simulink model "nao_linear_piloto_automatico"  (R2024a)
settings: Solver=VariableStepAuto  StartTime=0.0  StopTime=200  RelTol=1e-3
values from neighbouring files (symbols this model uses):
  Ka = 10    [NL_Parametros_Piloto_automatico.m]    (also in run_mil_export.m)
  TauA = 0.2    [NL_Parametros_Piloto_automatico.m]    (also in run_mil_export.m)
libraries: slpidlib x1, SignalEditorBlockLib x1
settings Model: Creator=kaiqu  LastModifiedBy=kaiqu

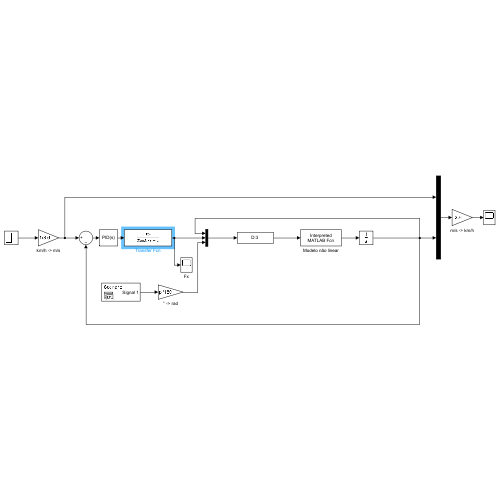
[thumbnail: Simulink's stored preview of the top-level diagram]
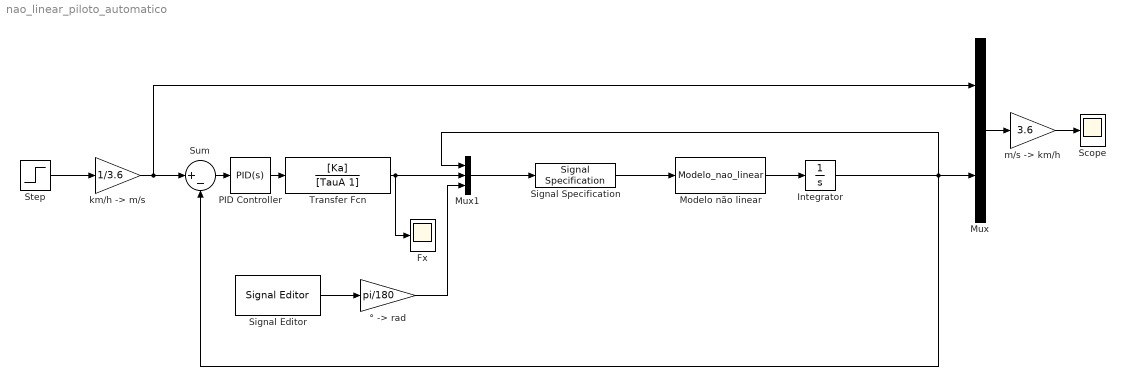
== system nao_linear_piloto_automatico ==
  Fx : Scope
  Integrator : Integrator  InitialCondition=50/3.6
  Modelo não linear : MATLABFcn  MATLABFcn=Modelo_nao_linear
  Mux : Mux  Inputs=2
  Mux1 : Mux  Inputs=3
  PID Controller : slpidlib/PID Controller  Controller=PID  Form=Parallel  TimeDomain=Continuous-time  UseExternalTs=off  SampleTime=-1  IntegratorMethod=Forward Euler  FilterMethod=Forward Euler  ControllerParametersSource=internal  P=477.204600781084  I=42.1664078975366  UseKiTs=off  D=178.763139862948  UseExternalDerivativeSource=off  N=1.8234120333855  UseFilter=on  TunerSelectOption=Transfer Function Based (PID Tuner App)  InitialConditionSource=internal  InitialConditionForIntegrator=0  InitialConditionForFilter=0  DifferentiatorICPrevScaledInput=0  ExternalReset=none  TrackingMode=off  Kt=1  LimitOutput=off  SatLimitsSource=internal  UpperSaturationLimit=inf  LowerSaturationLimit=-inf  LinearizeAsGain=on  AntiWindupMode=none  Kb=1  LimitIntegrator=off  UpperIntegratorSaturationLimit=inf  LowerIntegratorSaturationLimit=-inf  POutMin=[]  POutMax=[]  IOutMin=[]  IOutMax=[]  DOutMin=[]  DOutMax=[]  NOutMin=[]  NOutMax=[]  SumOutMin=[]  SumOutMax=[]  SaturationOutMin=[]  SaturationOutMax=[]  PParamMin=[]  PParamMax=[]  IParamMin=[]  IParamMax=[]  DParamMin=[]  DParamMax=[]  NParamMin=[]  NParamMax=[]  KbParamMin=[]  KbParamMax=[]  KtParamMin=[]  KtParamMax=[]  KbOutMin=[]  KbOutMax=[]  KtOutMin=[]  KtOutMax=[]  IntegratorOutMin=[]  IntegratorOutMax=[]  FilterOutMin=[]  FilterOutMax=[]  SumI1OutMin=[]  SumI1OutMax=[]  SumI2OutMin=[]  SumI2OutMax=[]  SumI3OutMin=[]  SumI3OutMax=[]  SumI4OutMin=[]  SumI4OutMax=[]  SumDOutMin=[]  SumDOutMax=[]  DifferentiatorOutMin=[]  DifferentiatorOutMax=[]  FilterDiffOutCoefMin=[]  FilterDiffOutCoefMax=[]  ReciprocalOutMin=[]  ReciprocalOutMax=[]  SumDenOutMin=[]  SumDenOutMax=[]  SumNumOutMin=[]  SumNumOutMax=[]  DivideOutMin=[]  DivideOutMax=[]  UdiffTsProdOutMin=[]  UdiffTsProdOutMax=[]  NTsProdOutMin=[]  NTsProdOutMax=[]  UintegralTsProdOutMin=[]  UintegralTsProdOutMax=[]  UngainTsProdOutMin=[]  UngainTsProdOutMax=[]  ClampingZeroOutDataTypeStr=Inherit: Inherit via back propagation  ClampingZeroOutMin=[]  ClampingZeroOutMax=[]  FilterDenConstantOutDataTypeStr=Inherit: Inherit via back propagation  FilterDenConstantOutMin=[]  FilterDenConstantOutMax=[]  PCopyOutDataTypeStr=Inherit: Inherit via back propagation  PCopyOutMin=[]  PCopyOutMax=[]  NCopyOutDataTypeStr=Inherit: Inherit via back propagation  NCopyOutMin=[]  NCopyOutMax=[]  IntegratorContinuousStateAttributes=''  IntegratorStateMustResolveToSignalObject=off  IntegratorRTWStateStorageClass=Auto  FilterContinuousStateAttributes=''  FilterStateMustResolveToSignalObject=off  FilterRTWStateStorageClass=Auto  ParallelPVariant=InternalParameters  IdealPVariant=Disabled  IVariant=InternalParameters  DVariant=InternalParameters  IntegratorVariant=Continuous  SatVariant=Disabled  AWVariant=Passthrough  PCopyVariant=Disabled  TRVariant=Disabled  FdbkBlocksVariant=Forward  IdealPFdbkVariant=Disabled  SatFdbkVariant=Disabled  DerivativeFilterVariant=ContFilter  NVariant=InternalParameters  NCopyVariant=Disabled  FilterICVariant=InternalICsFilter  IntegratorICVariant=InternalICs  ExternalResetVariant=Disabled  TRSumVariant=Passthrough  SumFdbkVariant=Disabled  SumVariant=Sum_PID  TsampFilterVariant=InternalTs  TsampNgainVariant=Passthrough  TsampIntegralVariant=Disabled_SignalSpec  ExternalSaturationOutDataTypeStr=Inherit: Same as second input  DerivativeSourceVariant=ErrorSignal
  Scope : Scope
  Signal Editor : SignalEditorBlockLib/Signal Editor  FileName=SINAL_RAMPA_1.mat  ActiveScenario=Scenario  ActiveSignal=Signal 1  IsBus=off  OutputBusObjectStr=Bus: BusObject  SampleTime=0  Interpolate=off  ZeroCross=off  OutputAfterFinalValue=Setting to zero  Unit=inherit  PreserveSignalName=on  ApplySigPropsToAllScenarios=on  ApplySigPropsToAllSignals=off
  Signal Specification : SignalSpecification  Dimensions=3
  Step : Step  Time=0  After=90  SampleTime=0
  Sum : Sum  Inputs=|+-
  Transfer Fcn : TransferFcn  Numerator=[Ka]  Denominator=[TauA 1]
  "km/h -> m/s" : Gain  Gain=1/3.6
  "m/s -> km/h" : Gain  Gain=3.6
  "° -> rad" : Gain  Gain=pi/180
  wires:
  Mux1/1 -> Signal Specification/1
  Modelo não linear/1 -> Integrator/1
  "m/s -> km/h"/1 -> Scope/1
  Mux/1 -> "m/s -> km/h"/1
  Integrator/1 -> Mux1/1, Mux/2, Sum/2
  Sum/1 -> PID Controller/1
  Step/1 -> "km/h -> m/s"/1
  "km/h -> m/s"/1 -> Mux/1, Sum/1
  Signal Editor/1 -> "° -> rad"/1
  "° -> rad"/1 -> Mux1/3
  PID Controller/1 -> Transfer Fcn/1
  Transfer Fcn/1 -> Fx/1, Mux1/2
  Signal Specification/1 -> Modelo não linear/1
